simulink model "MassSpringDamper"  (R2023b)
settings: Solver=VariableStepAuto  StartTime=0.0  StopTime=10.0  RelTol=1e-3
undefined symbols (not defined in the file): X, Y, Z
libraries: sm_lib x6, nesl_utility x4
settings Model: Creator=matte  LastModifiedBy=matte

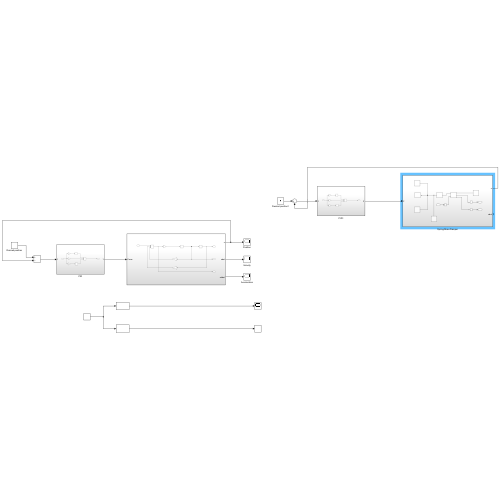
[thumbnail: Simulink's stored preview of the top-level diagram]
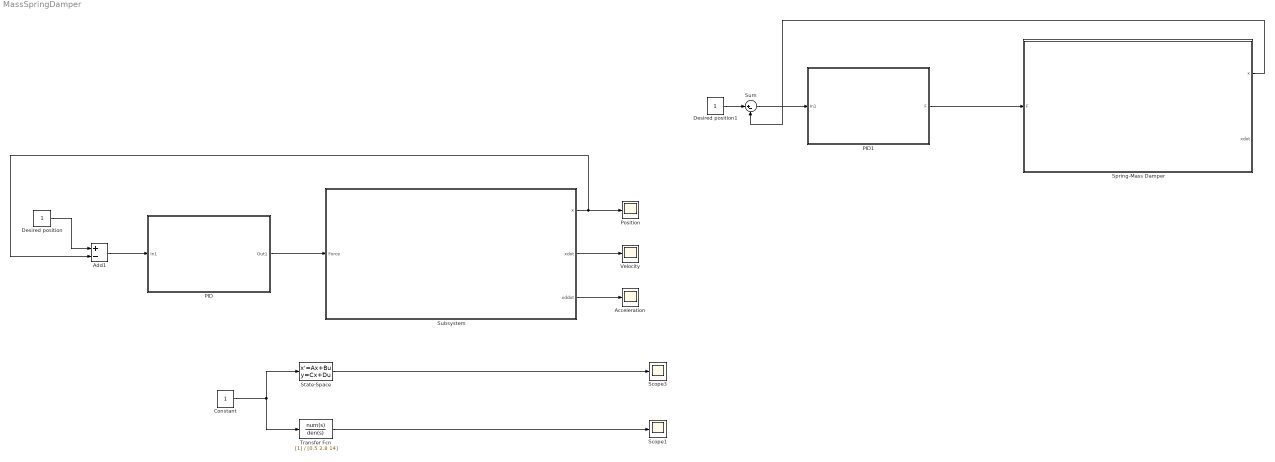
== system MassSpringDamper ==
  Acceleration : Scope
  Add1 : Sum  Inputs=+-
  Constant : Constant
  Desired position : Constant
  Desired position1 : Constant
  PID : Subsystem
  PID1 : Subsystem
  Position : Scope
  Scope1 : Scope
  Scope3 : Scope
  Spring-Mass Damper : Subsystem
  State-Space : StateSpace  A=[0 1; -14/0.5 -2.8/0.5]  B=[0; 2]  C=[1 0]  D=0  InitialCondition=0
  Subsystem : Subsystem
  Sum : Sum  Inputs=|+-
  Transfer Fcn : TransferFcn  Denominator=[0.5 2.8 14]
  Velocity : Scope
  wires:
  State-Space/1 -> Scope3/1
  Transfer Fcn/1 -> Scope1/1
  Subsystem/1(x) -> Position/1, Add1/2
  Desired position/1 -> Add1/1
  Constant/1 -> State-Space/1, Transfer Fcn/1
  Subsystem/2(xdot) -> Velocity/1
  Subsystem/3(xddot) -> Acceleration/1
  Desired position1/1 -> Sum/1
  Spring-Mass Damper/1(x) -> Sum/2
  Add1/1 -> PID/1(In1)
  PID/1(Out1) -> Subsystem/1(Force)
  Sum/1 -> PID1/1(In1)
  PID1/1(F) -> Spring-Mass Damper/1(F)

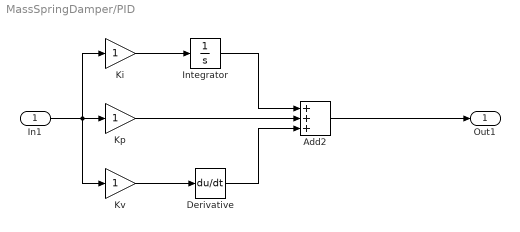
== system MassSpringDamper/PID ==
  In1 : Inport
  Add2 : Sum  Inputs=+++
  Derivative : Derivative
  Integrator : Integrator
  Ki : Gain
  Kp : Gain
  Kv : Gain
  Out1 : Outport
  wires:
  Ki/1 -> Integrator/1
  Kp/1 -> Add2/2
  Derivative/1 -> Add2/3
  In1/1 -> Kv/1, Ki/1, Kp/1
  Integrator/1 -> Add2/1
  Kv/1 -> Derivative/1
  Add2/1 -> Out1/1

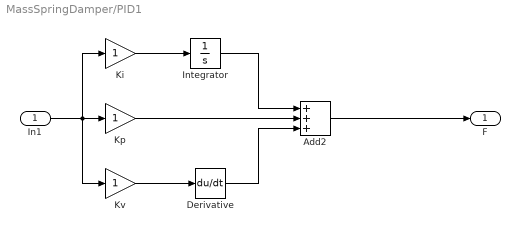
== system MassSpringDamper/PID1 ==
  In1 : Inport
  Add2 : Sum  Inputs=+++
  Derivative : Derivative
  Integrator : Integrator
  Ki : Gain
  Kp : Gain
  Kv : Gain
  F : Outport
  wires:
  Ki/1 -> Integrator/1
  Kp/1 -> Add2/2
  Derivative/1 -> Add2/3
  In1/1 -> Kv/1, Ki/1, Kp/1
  Integrator/1 -> Add2/1
  Kv/1 -> Derivative/1
  Add2/1 -> F/1

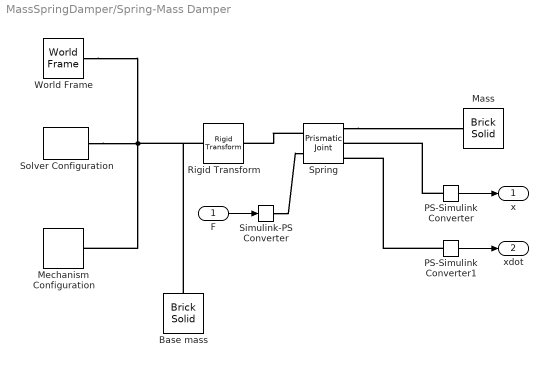
== system MassSpringDamper/Spring-Mass Damper ==
  F : Inport
  Base mass : sm_lib/Body Elements/Brick Solid  GraphicAmbientColor=[0.15 0.15 0.15 1.0]  BasedOnType=Mass  BrickDimensions=[1 1 1]  BrickDimensionsUnits=m  CenterOfMass=[0 0 0]  CenterOfMassUnits=m  GraphicDiffuseColor=[0.5 0.5 0.5]  Density=1000  DensityUnits=kg/m^3  DoExposeReferenceFrame=on  GraphicEmissiveColor=[0.0 0.0 0.0 1.0]  ExportEntireGeometry=off  SerializedFrames=<Frames/>  MarkerShape=Sphere  MarkerSize=10  GraphicType=FromGeometry  InertiaType=CalculateFromGeometry  Mass=1  MassUnits=kg  MomentsOfInertia=[1 1 1]  MomentsOfInertiaUnits=kg*m^2  GraphicOpacity=1.0  ProductsOfInertia=[0 0 0]  ProductsOfInertiaUnits=kg*m^2  GraphicShininess=75  GraphicSpecularColor=[0.5 0.5 0.5 1.0]  GraphicVisPropType=SimpleVisualProperties
  Mass : sm_lib/Body Elements/Brick Solid  GraphicAmbientColor=[0.15 0.15 0.15 1.0]  BasedOnType=Mass  BrickDimensions=[1 1 1]  BrickDimensionsUnits=m  CenterOfMass=[0 0 0]  CenterOfMassUnits=m  GraphicDiffuseColor=[0.5 0.5 0.5]  Density=1000  DensityUnits=kg/m^3  DoExposeReferenceFrame=on  GraphicEmissiveColor=[0.0 0.0 0.0 1.0]  ExportEntireGeometry=off  SerializedFrames=<Frames/>  MarkerShape=Sphere  MarkerSize=10  GraphicType=FromGeometry  InertiaType=CalculateFromGeometry  Mass=1  MassUnits=kg  MomentsOfInertia=[1 1 1]  MomentsOfInertiaUnits=kg*m^2  GraphicOpacity=1.0  ProductsOfInertia=[0 0 0]  ProductsOfInertiaUnits=kg*m^2  GraphicShininess=75  GraphicSpecularColor=[0.5 0.5 0.5 1.0]  GraphicVisPropType=SimpleVisualProperties
  Mechanism Configuration : sm_lib/Utilities/Mechanism Configuration  UniformGravity=Constant  GravityVector=[0 0 -9.80665]  GravityVectorUnits=m/s^2  LinearizationDelta=0.001  JointModeTransitionNonlinearIterations=2
  PS-Simulink Converter : nesl_utility/PS-Simulink Converter  PhysicalDomain=network_engine_domain  SubClassName=ps_output  LeftPortType=input  RightPortType=output  PseudoPeriodic=off  Frequencies=[]  VectorFormat=inherit  Unit=inherit  AffineConversion=off
  PS-Simulink Converter1 : nesl_utility/PS-Simulink Converter  PhysicalDomain=network_engine_domain  SubClassName=ps_output  LeftPortType=input  RightPortType=output  PseudoPeriodic=off  Frequencies=[]  VectorFormat=inherit  Unit=inherit  AffineConversion=off
  Rigid Transform : sm_lib/Frames and Transforms/Rigid Transform  TranslationMethod=StandardAxis  TranslationStandardOffset=15  TranslationStandardOffsetUnits=cm  TranslationStandardAxis=+X  TranslationCartesianOffset=[0 0 0]  TranslationCartesianOffsetUnits=m  TranslationROffset=0  TranslationROffsetUnits=m  TranslationZOffset=0  TranslationZOffsetUnits=m  TranslationThetaOffset=0  TranslationThetaOffsetUnits=deg  RotationMethod=StandardAxis  RotationAngleUnits=deg  RotationStandardAxis=+Y  RotationAngle=90  RotationArbitraryAxis=[0 0 1]  FollAlignAxisA=+X  BaseAlignAxisA=+Y  FollAlignAxisB=+Y  BaseAlignAxisB=+Z  RotationSequenceAxes=FollowerAxes  RotationSequence=XYX  RotationSequenceAngles=[0 0 0]  RotationSequenceAnglesUnits=deg  RotationMatrix=[1 0 0; 0 1 0; 0 0 1]  Quaternion=[1 0 0 0]
  Simulink-PS Converter : nesl_utility/Simulink-PS Converter  PhysicalDomain=network_engine_domain  SubClassName=ps_input  LeftPortType=input  RightPortType=output  PseudoPeriodic=off  Frequencies=[]  NoiseDistribution=none  NoiseParameters=[]  Unit=1  AffineConversion=off  FilteringAndDerivatives=provide  SimscapeFilterOrder=1  InputFilterTimeConstant=0.001  UdotUserProvided=0
  Solver Configuration : nesl_utility/Solver Configuration  PhysicalDomain=network_engine_domain  SubClassName=solver  LeftPortType=input  RightPortType=generic  Tones=[]  Harmonics=[]  SimulateNoise=off  Profile=off  UseLocalSampling=off  EnableSwitchedLinearOptims=on  FrequencyDomain=off  UseCCode=off  RelTol=0.001  AbsTol=1e-06  MinStep=1e-09  ToWorkspace=off  RevertToSquareIcSolve=off  NumHomotopyIterations=100  PhasorMode=off  PhasorModeNumHarmonics=1  ConsistencySolver=NEWTON_XTOL_AFTER_FTOL  IndexReductionMethod=DerivativeReplacement  DoDC=off  ResidualTolerance=1e-09  ConsistencyTolSource=GLOBAL  ConsistencyAbsTol=0.001  ConsistencyRelTol=0.001  ConsistencyTolFactor=0.001  UseLocalSolver=off  LocalSolverChoice=NE_BACKWARD_EULER_ADVANCER  ResolveIndetEquations=on  FunctionEvalNumThread=1  LocalSolverSampleTime=0.001  DoFixedCost=off  MaxNonlinIter=3  MaxModeIter=2  ComputeImpulses=off  ImpulseIterations=2  LinearAlgebra=auto  LinearAlgebraNumThread=0  EquationFormulation=NE_TIME_EF  DelaysMemoryBudget=1024  AutomaticFiltering=on  FilteringTimeConstant=0.001  PartitionStorageMethod=AS_NEEDED  PartitionMemoryBudget=1024  PartitionMethod=ROBUST  MultibodyUseLocalSolver=off  MultibodyLocalSolverChoice=ODE1  MultibodyLocalSolverSampleTime=0.001
  Spring : sm_lib/Joints/Prismatic Joint  JointMode=Normal  SenseConstraintForce=off  SenseConstraintForceX=off  SenseConstraintForceY=off  SenseConstraintForceZ=off  SenseConstraintTorque=off  SenseConstraintTorqueX=off  SenseConstraintTorqueY=off  SenseConstraintTorqueZ=off  SenseTotalForce=off  SenseTotalForceX=off  SenseTotalForceY=off  SenseTotalForceZ=off  SenseTotalTorque=off  SenseTotalTorqueX=off  SenseTotalTorqueY=off  SenseTotalTorqueZ=off  CompositeWrenchDir=FollowerOnBase  CompositeWrenchFrame=BaseFrame  EquilibriumPosition=10  EquilibriumPositionUnits=cm  SpringStiffness=20  SpringStiffnessUnits=N/m  DampingCoefficient=2.8  DampingCoefficientUnits=N/(m/s)  TorqueActuationMode=InputTorque  MotionActuationMode=ComputedMotion  SensePosition=on  SenseVelocity=on  SenseAcceleration=off  SenseTorqueForce=off  SenseLowerLimitTorqueForce=off  SenseUpperLimitTorqueForce=off  LowerLimitSpecify=off  LowerLimitBound=-1  LowerLimitBoundUnits=m  LowerLimitStiffness=1e6  LowerLimitStiffnessUnits=N/m  LowerLimitDamping=1e3  LowerLimitDampingUnits=N/(m/s)  LowerLimitTransitionRegionWidth=1e-4  LowerLimitTransitionRegionWidthUnits=m  UpperLimitSpecify=off  UpperLimitBound=1  UpperLimitBoundUnits=m  UpperLimitStiffness=1e6  UpperLimitStiffnessUnits=N/m  UpperLimitDamping=1e3  UpperLimitDampingUnits=N/(m/s)  UpperLimitTransitionRegionWidth=1e-4  UpperLimitTransitionRegionWidthUnits=m  PositionTargetSpecify=off  PositionTargetPriority=High  PositionTargetValue=0  PositionTargetValueUnits=m  VelocityTargetSpecify=off  VelocityTargetPriority=High  VelocityTargetValue=0  VelocityTargetValueUnits=m/s
  World Frame : sm_lib/Frames and Transforms/World Frame
  x : Outport
  xdot : Outport  Port=2
  wires:
  PS-Simulink Converter/1 -> x/1
  F/1 -> Simulink-PS Converter/1
  PS-Simulink Converter1/1 -> xdot/1
  connections:
  World Frame/RConn1 -- Solver Configuration/RConn1 -- Mechanism Configuration/RConn1 -- Rigid Transform/LConn1 -- Base mass/RConn1
  Spring/LConn1 -- Rigid Transform/RConn1
  PS-Simulink Converter/LConn1 -- Spring/RConn2
  PS-Simulink Converter1/LConn1 -- Spring/RConn3
  Simulink-PS Converter/RConn1 -- Spring/LConn2
  Spring/RConn1 -- Mass/RConn1

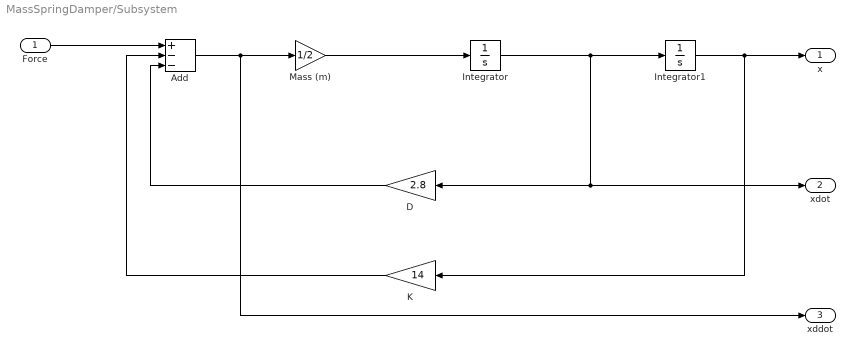
== system MassSpringDamper/Subsystem ==
  Force : Inport
  Add : Sum  Inputs=+--
  D : Gain  Gain=2.8
  Integrator : Integrator
  Integrator1 : Integrator
  K : Gain  Gain=14
  Mass (m) : Gain  Gain=1/2
  x : Outport
  xdot : Outport  Port=2
  xddot : Outport  Port=3
  wires:
  Integrator1/1 -> x/1, K/1
  Integrator/1 -> Integrator1/1, xdot/1, D/1
  Mass (m)/1 -> Integrator/1
  Add/1 -> xddot/1, Mass (m)/1
  D/1 -> Add/3
  Force/1 -> Add/1
  K/1 -> Add/2
